simulink model "ball_impact"  (Simulink 8.1)
settings: Solver=ode4  SolverMode=SingleTasking  StartTime=0.0  StopTime=inf  FixedStep=0.0005  RelTol=1e-3
StartFcn:
  |  warndlg('Dexterit-E models cannot run under simulation. Please compile your model and run it from within Dexterit-E.');set_param(bdroot,'SimulationCommand','stop')
undefined symbols (not defined in the file or in its folder): CreateParameterTableGUI, slselsubs
libraries: xpclib x30, simulink x8, KINARM_general x3, KINARM_loads x2, Video x2, KINARM_EP_loads x1
(part 3 of 5)

== system ball_impact/Parameter Table Defn/events ==
  E_BALL_RELEASE;BALL_RELEASE;;Ball released at the slope top;;;none;; : Constant
  E_CONTACT_END;CONTACT_END;;Ball-hand contact ended;;;none;; : Constant  Value=3
  E_CONTACT_START;CONTACT_START;;Ball-hand contact started (pen greater than 0);;;none;; : Constant  Value=2
  E_HAND_LEFT_HOME;HAND_LEFT_HOME;;Hand left home before impact - trial aborted;;;error;; : Constant  Value=4
  Terminator{1..4} (4 alike) : Terminator
  wires:
  E_BALL_RELEASE;BALL_RELEASE;;Ball released at the slope top;;;none;;/1 -> Terminator1/1
  E_CONTACT_START;CONTACT_START;;Ball-hand contact started (pen greater than 0);;;none;;/1 -> Terminator2/1
  E_CONTACT_END;CONTACT_END;;Ball-hand contact ended;;;none;;/1 -> Terminator3/1
  E_HAND_LEFT_HOME;HAND_LEFT_HOME;;Hand left home before impact - trial aborted;;;error;;/1 -> Terminator4/1

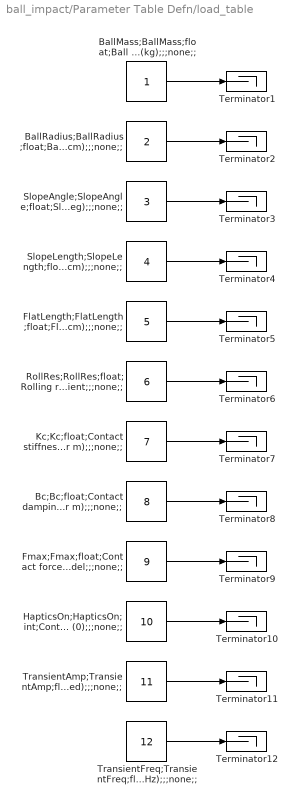
== system ball_impact/Parameter Table Defn/load_table ==
  BallMass;BallMass;float;Ball mass (kg);;;none;; : Constant
  BallRadius;BallRadius;float;Ball radius (cm);;;none;; : Constant  Value=2
  Bc;Bc;float;Contact damping (N s per m);;;none;; : Constant  Value=8
  FlatLength;FlatLength;float;Flat run-out length (cm);;;none;; : Constant  Value=5
  "Fmax;Fmax;float;Contact force clamp (N), also hard-clamped in the model;;;none;;" : Constant  Value=9
  HapticsOn;HapticsOn;int;Contact force on (1) or visual only (0);;;none;; : Constant  Value=10
  Kc;Kc;float;Contact stiffness (N per m);;;none;; : Constant  Value=7
  RollRes;RollRes;float;Rolling resistance coefficient;;;none;; : Constant  Value=6
  SlopeAngle;SlopeAngle;float;Slope angle (deg);;;none;; : Constant  Value=3
  SlopeLength;SlopeLength;float;Slope length (cm);;;none;; : Constant  Value=4
  Terminator{1..12} (12 alike) : Terminator
  TransientAmp;TransientAmp;float;Impact transient amplitude (N per unit impact speed);;;none;; : Constant  Value=11
  TransientFreq;TransientFreq;float;Impact transient frequency (Hz);;;none;; : Constant  Value=12
  wires:
  BallMass;BallMass;float;Ball mass (kg);;;none;;/1 -> Terminator1/1
  BallRadius;BallRadius;float;Ball radius (cm);;;none;;/1 -> Terminator2/1
  SlopeAngle;SlopeAngle;float;Slope angle (deg);;;none;;/1 -> Terminator3/1
  SlopeLength;SlopeLength;float;Slope length (cm);;;none;;/1 -> Terminator4/1
  FlatLength;FlatLength;float;Flat run-out length (cm);;;none;;/1 -> Terminator5/1
  RollRes;RollRes;float;Rolling resistance coefficient;;;none;;/1 -> Terminator6/1
  Kc;Kc;float;Contact stiffness (N per m);;;none;;/1 -> Terminator7/1
  Bc;Bc;float;Contact damping (N s per m);;;none;;/1 -> Terminator8/1
  "Fmax;Fmax;float;Contact force clamp (N), also hard-clamped in the model;;;none;;"/1 -> Terminator9/1
  HapticsOn;HapticsOn;int;Contact force on (1) or visual only (0);;;none;;/1 -> Terminator10/1
  TransientAmp;TransientAmp;float;Impact transient amplitude (N per unit impact speed);;;none;;/1 -> Terminator11/1
  TransientFreq;TransientFreq;float;Impact transient frequency (Hz);;;none;;/1 -> Terminator12/1

== system ball_impact/Parameter Table Defn/target_table ==
  Colour;Colour;colour;Target colour;;;none;; : Constant  Value=5
  LogRadius;LogRadius;float;Hand-in-target logical radius (cm);;;none;; : Constant  Value=4
  Terminator{1..5} (5 alike) : Terminator
  VisRadius;VisRadius;float;Drawn radius of the target circle (cm);;;none;; : Constant  Value=3
  col_x;X;float;X Position (cm) of the target relative to  local (0,0);;;none;; : Constant
  col_y;Y;float;Y Position (cm) of the target relative to  local (0,0);;;none;; : Constant  Value=2
  wires:
  col_x;X;float;X Position (cm) of the target relative to  local (0,0);;;none;;/1 -> Terminator1/1
  col_y;Y;float;Y Position (cm) of the target relative to  local (0,0);;;none;;/1 -> Terminator2/1
  VisRadius;VisRadius;float;Drawn radius of the target circle (cm);;;none;;/1 -> Terminator3/1
  LogRadius;LogRadius;float;Hand-in-target logical radius (cm);;;none;;/1 -> Terminator4/1
  Colour;Colour;colour;Target colour;;;none;;/1 -> Terminator5/1

== system ball_impact/Parameter Table Defn/task_definition ==
  INSTRUCTIONS= : Constant
  LOAD_FOR=EITHER : Constant  Value=2
  Terminator1 : Terminator
  Terminator2 : Terminator
  wires:
  INSTRUCTIONS=/1 -> Terminator1/1
  LOAD_FOR=EITHER/1 -> Terminator2/1

== system ball_impact/Parameter Table Defn/task_wide ==
  ApproachDir;ApproachDir;float;Ball approach direction (deg) with 90 = lateral from +X and 0 = toward body;;;none;; : Constant  Value=2
  HandRadius;HandRadius;float;Hand contact (paddle) radius (cm);;;none;; : Constant
  Terminator1 : Terminator
  Terminator2 : Terminator
  wires:
  HandRadius;HandRadius;float;Hand contact (paddle) radius (cm);;;none;;/1 -> Terminator1/1
  ApproachDir;ApproachDir;float;Ball approach direction (deg) with 90 = lateral from +X and 0 = toward body;;;none;;/1 -> Terminator2/1

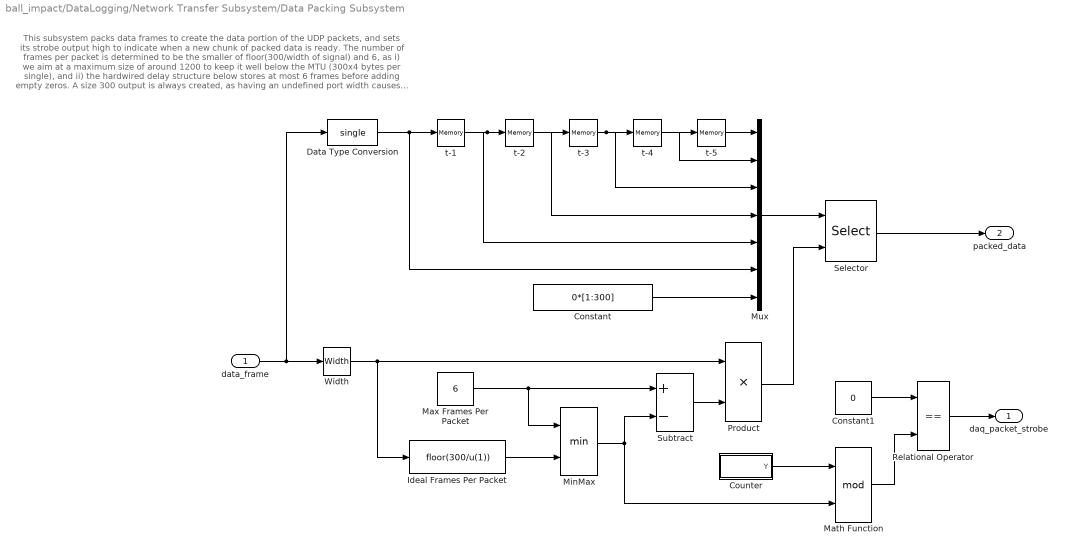
== system ball_impact/DataLogging/Network Transfer Subsystem/Data Packing Subsystem ==
  note: This subsystem packs data frames to create the data portion of the UDP packets, and sets its strobe output high to indicate when a
      | new chunk of packed data is ready. The number of frames per packet is determined to be the smaller of floor(300/width of signal)
      | and 6, as i) we aim at a maximum size of around 1200 to keep it well below the MTU (300x4 bytes per single), and ii) the hardwired
      | delay structure below stores at most 6 frames before adding empty zeros. A size 300 output is always created, as having an undefined
      | port width causes Simulink problems.
  data_frame : Inport
  Constant : Constant  Value=0*[1:300]  OutDataTypeStr=single
  Constant1 : Constant  Value=0
  Counter : Subsystem
  Data Type Conversion : DataTypeConversion  OutDataTypeStr=single  SaturateOnIntegerOverflow=on  RndMeth=Zero
  Ideal Frames Per Packet : Fcn  Expr=floor(300/u(1))
  Math Function : Math  Operator=mod  SaturateOnIntegerOverflow=on
  Max Frames Per Packet : Constant  Value=6
  MinMax : MinMax  Inputs=2
  Mux : Mux  Inputs=7
  Product : Product  RndMeth=Zero
  Relational Operator : RelationalOperator  Operator===  OutDataTypeStr=boolean
  Selector : Selector  IndexMode=Zero-based  IndexOptions=Starting index (port)  Indices=[1:300]  OutputSizes=[([([([([(300)])])])])]
  Subtract : Sum  Inputs=+-
  Width : Width
  t-{1..5} (5 alike) : Memory  InheritSampleTime=on
  daq_packet_strobe : Outport
  packed_data : Outport  Port=2
  wires:
  Ideal Frames Per Packet/1 -> MinMax/2
  Width/1 -> Ideal Frames Per Packet/1, Product/1
  Product/1 -> Selector/2
  Subtract/1 -> Product/2
  Max Frames Per Packet/1 -> MinMax/1, Subtract/1
  MinMax/1 -> Subtract/2, Math Function/2
  Constant/1 -> Mux/7
  Selector/1 -> packed_data/1
  Mux/1 -> Selector/1
  t-5/1 -> Mux/1
  Data Type Conversion/1 -> Mux/6, t-1/1
  t-3/1 -> Mux/3, t-4/1
  t-4/1 -> Mux/2, t-5/1
  t-2/1 -> Mux/4, t-3/1
  t-1/1 -> Mux/5, t-2/1
  Math Function/1 -> Relational Operator/2
  Constant1/1 -> Relational Operator/1
  Relational Operator/1 -> daq_packet_strobe/1
  Counter/1(Y) -> Math Function/1
  data_frame/1 -> Data Type Conversion/1, Width/1

== system ball_impact/DataLogging/Network Transfer Subsystem/UDP Send Subsystem ==
  packet_data : Inport
  Trigger : TriggerPort  TriggerType=function-call
  Counter Free-Running : simulink/Sources/Counter Free-Running  NumBits=32  tsamp=-1
  Pack : xpclib/UDP/Pack  datatypes={'single'}  byteAlign=1
  Send : xpclib/UDP/Send  ipAddress=192.168.0.1  ipPort=50000  localPort=50000  vblLen=off  sampletime=-1
  total_packets_sent : Outport  InitialOutput=0
  wires:
  packet_data/1 -> Pack/1
  Pack/1 -> Send/1
  Counter Free-Running/1 -> total_packets_sent/1

== system ball_impact/DataLogging/Poll Force Plates/plate1 ==
  send_packet : Inport
  gain : Inport  Port=2
  calib_matrix : Inport  Port=3
  ain_slope : Inport  Port=4
  ain_offset : Inport  Port=5
  orientation : Inport  Port=6
  zero_voltage : Inport  Port=7
  Enable : EnablePort
  Receive : xpclib/UDP/Receive  ipAddress=192.168.0.101  ipPort=53795  width=64  vblLen=off  sampletime=BKIN_STEP_TIME
  Send : xpclib/UDP/Send  ipAddress=192.168.0.101  ipPort=52360  localPort=53795  vblLen=off  sampletime=0.0005
  Terminator : Terminator
  parse packet 1 : MATLAB Function  TreatAsAtomicUnit=on
  Forces P1 : Outport
  Moments P1 : Outport  Port=2
  Timer P1 : Outport  Port=3
  wires:
  send_packet/1 -> Send/1
  parse packet 1/3(timer) -> Timer P1/1
  Receive/2 -> Terminator/1
  gain/1 -> parse packet 1/3(gain)
  Receive/1 -> parse packet 1/1(packet)
  calib_matrix/1 -> parse packet 1/2(calibration)
  parse packet 1/1(forces) -> Forces P1/1
  parse packet 1/2(moments) -> Moments P1/1
  ain_offset/1 -> parse packet 1/5(ain_offset)
  ain_slope/1 -> parse packet 1/4(ain_slope)
  orientation/1 -> parse packet 1/6(orientation)
  zero_voltage/1 -> parse packet 1/7(zero_voltage)

== system ball_impact/DataLogging/Poll Force Plates/plate2 ==
  send_packet : Inport
  gain : Inport  Port=2
  calib_matrix : Inport  Port=3
  ain_slope : Inport  Port=4
  ain_offset : Inport  Port=5
  orientation : Inport  Port=6
  zero_voltage : Inport  Port=7
  Enable : EnablePort
  Receive1 : xpclib/UDP/Receive  ipAddress=192.168.0.102  ipPort=53796  width=64  vblLen=off  sampletime=BKIN_STEP_TIME
  Send1 : xpclib/UDP/Send  ipAddress=192.168.0.102  ipPort=52360  localPort=53796  vblLen=off  sampletime=0.0005
  Terminator : Terminator
  parse packet 1 : MATLAB Function  TreatAsAtomicUnit=on
  Forces P1 : Outport
  Moments P1 : Outport  Port=2
  Timer P1 : Outport  Port=3
  wires:
  send_packet/1 -> Send1/1
  parse packet 1/3(timer) -> Timer P1/1
  Receive1/2 -> Terminator/1
  gain/1 -> parse packet 1/3(gain)
  Receive1/1 -> parse packet 1/1(packet)
  calib_matrix/1 -> parse packet 1/2(calibration)
  parse packet 1/1(forces) -> Forces P1/1
  parse packet 1/2(moments) -> Moments P1/1
  ain_offset/1 -> parse packet 1/5(ain_offset)
  ain_slope/1 -> parse packet 1/4(ain_slope)
  orientation/1 -> parse packet 1/6(orientation)
  zero_voltage/1 -> parse packet 1/7(zero_voltage)

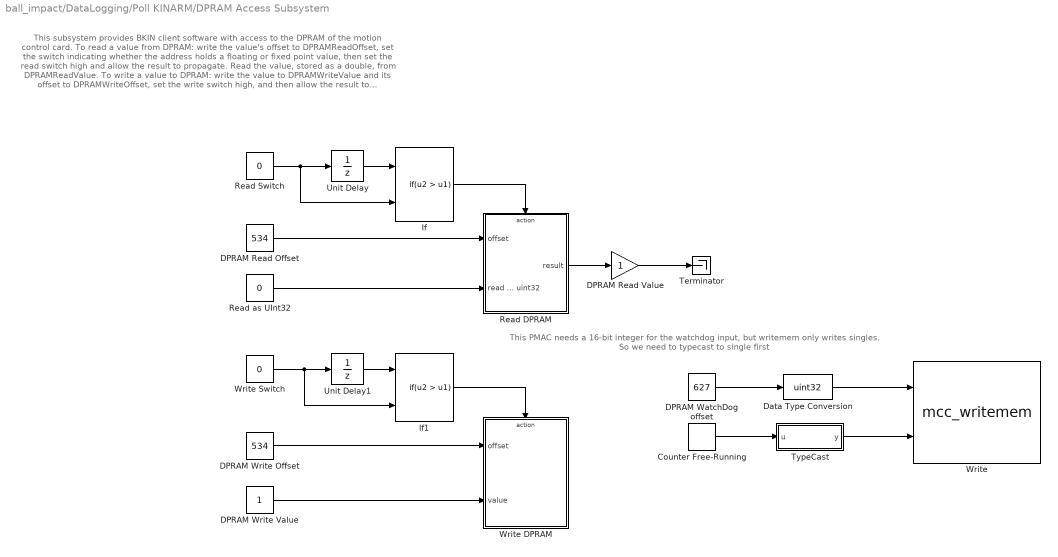
== system ball_impact/DataLogging/Poll KINARM/DPRAM Access Subsystem ==
  note: This PMAC needs a 16-bit integer for the watchdog input, but writemem
      | only writes singles.  So we need to typecast to single first
  note: This subsystem provides BKIN client software with access to the DPRAM of the motion control card.
      |
      | To read a value from DPRAM: write the value's offset to DPRAMReadOffset, set the switch indicating
      | whether the address holds a floating or fixed point value, then set the read switch high and allow the
      | result to propagate. Read the value, stored as a double, from DPRAMReadValue.
      |
      | To write a value to DPRAM: write the value to DPRAMWriteValue and its offset to DPRAMWriteOffset,
      | set the write switch high, and then allow the result to propagate. There is currently no option to write
      | values as UInt32s, akin to that for reading values.
      |
      | The default value for the offsets (0x216) is the lowest meaningful offset, the PLC switch variable.
  Counter Free-Running : simulink/Sources/Counter Free-Running  NumBits=16  tsamp=-1
  DPRAM Read Offset : Constant  Value=534  OutDataTypeStr=double
  DPRAM Read Value : Gain  SaturateOnIntegerOverflow=on  OutDataTypeStr=Inherit: Same as input  ParamDataTypeStr=Inherit: Same as input
  DPRAM WatchDog offset : Constant  Value=627  OutDataTypeStr=double
  DPRAM Write Offset : Constant  Value=534  OutDataTypeStr=double
  DPRAM Write Value : Constant
  Data Type Conversion : DataTypeConversion  OutDataTypeStr=uint32  SaturateOnIntegerOverflow=on  RndMeth=Zero
  If : If  NumInputs=2  IfExpression=u2 > u1  ShowElse=off
  If1 : If  NumInputs=2  IfExpression=u2 > u1  ShowElse=off
  Read DPRAM : Subsystem  TreatAsAtomicUnit=on
  Read Switch : Constant  Value=0
  Read as UInt32 : Constant  Value=0  OutDataTypeStr=double
  Terminator : Terminator
  TypeCast : MATLAB Function  TreatAsAtomicUnit=on
  Unit Delay : UnitDelay  SampleTime=-1
  Unit Delay1 : UnitDelay  SampleTime=-1
  Write : S-Function  Priority=6  FunctionName=mcc_writemem  EnableBusSupport=off
  Write DPRAM : Subsystem  TreatAsAtomicUnit=on
  Write Switch : Constant  Value=0
  wires:
  TypeCast/1(y) -> Write/2
  DPRAM Write Offset/1 -> Write DPRAM/1(offset)
  DPRAM Write Value/1 -> Write DPRAM/2(value)
  If1/1 -> Write DPRAM/Action
  Write Switch/1 -> Unit Delay1/1, If1/2
  DPRAM Read Value/1 -> Terminator/1
  Read DPRAM/1(result) -> DPRAM Read Value/1
  If/1 -> Read DPRAM/Action
  DPRAM Read Offset/1 -> Read DPRAM/1(offset)
  Read Switch/1 -> Unit Delay/1, If/2
  Unit Delay/1 -> If/1
  Unit Delay1/1 -> If1/1
  Read as UInt32/1 -> Read DPRAM/2(read as uint32)
  Data Type Conversion/1 -> Write/1
  DPRAM WatchDog offset/1 -> Data Type Conversion/1
  Counter Free-Running/1 -> TypeCast/1(u)

== system ball_impact/DataLogging/Poll KINARM/Force Sensor Control Subsystem ==
  note: This subsystem receives data from force sensors in the KINARM setup, and starts and stops the data transfer in response to changes in
      | the force sensor parameters in the system above. Each KINARM EP can have a force sensor, so there can currently be up to two in a
      | given setup. The force sensors transmit data over UDP, and parameters of the data transfer (such as the data rate and IP address) are
      | configured for each force sensor individually via a web interface they provide. BKIN preconfigures force sensors with IP addresses
      | 192.168.0.10-11, where the first address is given to the sensor for robot 1 and the second to that for robot 2.
  note: Each subsystem also handles the receiving of data from its particular sensor. When a sensor is indicated as present, the latest data from
      | its IP is unpacked and placed into a 1x6 array (zeros are explicitly specified when a sensor is indicated as not present). The arrays for
      | the individual sensors are combined into a 2x6 matrix, similar to how robot data is handled in the system above.
      |
      | Each packet received from a force sensor contains the following:
      |      sequence number [uint32]
      |      internal sequence number [uint32]
      |      system status code [uint32]
      |      x-axis force [int32]
      |      y-axis force [int32]
      |      z-axis force [int32]
      |      x-axis torque [int32]
      |      y-axis torque [int32]
      |      z-axis torque [int32]
      |
      | For more information, again see the ATI Net Interface guide.
  note: Each "force sensor x" subsystem here starts and stops the data transfer from its respective force sensor. When the input flag indicating
      | the presence (1: yes, 0: no) of a force sensor changes, the respective subsystem sends a command message via UDP to that force
      | sensor's IP address that starts or stops the data transfer accordingly. For details about the structure of the command message, see the
      | ATI Net Interface guide.
      |
      | Note that the default setting for all force sensors is 1, for "present", in the system above. This is done so that whenever BKIN's client
      | software applies hardware settings to a task program, it must first lower all force sensor flags and then raise those for whichever sensors
      | are present again. This forces all sensors off in case they were not stopped properly by a previous task. This would not stop data that
      | had been transmitted from being received, so when a force sensor is marked as not present the data is zeroed explicitly.
  Robot 1 Force Sensor : Inport
  Robot 2 Force Sensor : Inport  Port=2
  Force Sensor 1 Subsystem : Subsystem
  Force Sensor 2 Subsystem : Subsystem
  Mux8 : Mux  Inputs=2
  Force Sensor Data : Outport
  wires:
  Robot 1 Force Sensor/1 -> Force Sensor 1 Subsystem/1(Force Sensor 1 Present)
  Robot 2 Force Sensor/1 -> Force Sensor 2 Subsystem/1(Force Sensor 2 Present)
  Force Sensor 1 Subsystem/1(Out1) -> Mux8/1
  Force Sensor 2 Subsystem/1(Out1) -> Mux8/2
  Mux8/1 -> Force Sensor Data/1

== system ball_impact/DataLogging/Poll KINARM/Terminators for Gotos ==
  Terminator{,1..4} (5 alike) : Terminator
  wires:
  [primary_encoder_data] -> Terminator/1
  [robot1_motor_parameters] -> Terminator1/1
  [robot2_motor_parameters] -> Terminator2/1
  [robot1_calibration_parameters] -> Terminator3/1
  [robot2_calibration_parameters] -> Terminator4/1

== system ball_impact/DataLogging/Network Transfer Subsystem/Data Packing Subsystem/Counter ==
  Constant : Constant
  Sum : Sum  Inputs=|++  SaturateOnIntegerOverflow=on
  Unit Delay : UnitDelay  SampleTime=-1
  Y : Outport
  wires:
  Constant/1 -> Sum/2
  Sum/1 -> Unit Delay/1, Y/1
  Unit Delay/1 -> Sum/1

== system ball_impact/DataLogging/Poll KINARM/DPRAM Access Subsystem/Read DPRAM ==
  offset : Inport
  read as uint32 : Inport  Port=2
  Action Port : ActionPort
  Data Type Conversion : DataTypeConversion  OutDataTypeStr=uint32  SaturateOnIntegerOverflow=on  RndMeth=Zero
  Data Type Conversion1 : DataTypeConversion  OutDataTypeStr=double  SaturateOnIntegerOverflow=on  RndMeth=Zero
  Data Type Conversion2 : DataTypeConversion  OutDataTypeStr=uint32  SaturateOnIntegerOverflow=on  RndMeth=Zero
  Mux : Mux  Inputs=2
  Read : S-Function  Priority=6  FunctionName=mcc_readmem  EnableBusSupport=off
  result : Outport
  wires:
  Data Type Conversion/1 -> Mux/1
  Data Type Conversion1/1 -> result/1
  Read/1 -> Data Type Conversion1/1
  offset/1 -> Data Type Conversion/1
  read as uint32/1 -> Data Type Conversion2/1
  Data Type Conversion2/1 -> Mux/2
  Mux/1 -> Read/1

== system ball_impact/DataLogging/Poll KINARM/DPRAM Access Subsystem/Write DPRAM ==
  offset : Inport
  value : Inport  Port=2
  Action Port : ActionPort
  Data Type Conversion : DataTypeConversion  OutDataTypeStr=uint32  SaturateOnIntegerOverflow=on  RndMeth=Zero
  Data Type Conversion1 : DataTypeConversion  OutDataTypeStr=single  SaturateOnIntegerOverflow=on  RndMeth=Zero
  Write : S-Function  Priority=6  FunctionName=mcc_writemem  EnableBusSupport=off
  wires:
  Data Type Conversion1/1 -> Write/2
  Data Type Conversion/1 -> Write/1
  offset/1 -> Data Type Conversion/1
  value/1 -> Data Type Conversion1/1

== system ball_impact/DataLogging/Poll KINARM/Force Sensor Control Subsystem/Force Sensor 1 Subsystem ==
  Force Sensor 1 Present : Inport
  Byte Reversal : xpclib/UDP/Byte Reversal  numInp=1
  Byte Reversal1 : xpclib/UDP/Byte Reversal  numInp=1
  Constant : Constant  Value=zeros(1, 7);  OutDataTypeStr=double
  Create timestamp : MATLAB Function  TreatAsAtomicUnit=on
  Data Type Conversion : DataTypeConversion
  Detect Change : simulink/Logic and Bit Operations/Detect Change  vinit=1  InputProcessing=Inherited  OutDataTypeStr=uint8
  If Action Subsystem : Subsystem  TreatAsAtomicUnit=on
  Mux : Mux  Inputs=2
  Receive from Robot 1 Force Sensor : xpclib/UDP/Receive  ipAddress=192.168.0.10  ipPort=51000  width=36  vblLen=off  sampletime=BKIN_STEP_TIME
  Switch : Switch  Criteria=u2 > Threshold
  Terminator : Terminator
  Unpack : xpclib/UDP/Unpack  dimensions={3, 6}  datatypes={'uint32', 'int32'}  byteAlign=1
  Out1 : Outport
  wires:
  Receive from Robot 1 Force Sensor/1 -> Unpack/1
  Receive from Robot 1 Force Sensor/2 -> Terminator/1
  Force Sensor 1 Present/1 -> Switch/2, If Action Subsystem/1(In1), Detect Change/1
  Constant/1 -> Switch/3
  Switch/1 -> Out1/1
  Unpack/2 -> Byte Reversal/1
  Unpack/1 -> Byte Reversal1/1
  Byte Reversal/1 -> Data Type Conversion/1
  Detect Change/1 -> If Action Subsystem/Enable
  Create timestamp/1(timestamp_out) -> Mux/2
  Data Type Conversion/1 -> Mux/1
  Mux/1 -> Switch/1
  Byte Reversal1/1 -> Create timestamp/1(times_in)

== system ball_impact/DataLogging/Poll KINARM/Force Sensor Control Subsystem/Force Sensor 2 Subsystem ==
  Force Sensor 2 Present : Inport
  Byte Reversal : xpclib/UDP/Byte Reversal  numInp=1
  Byte Reversal1 : xpclib/UDP/Byte Reversal  numInp=1
  Constant1 : Constant  Value=zeros(1, 7);  OutDataTypeStr=double
  Create timestamp : MATLAB Function  TreatAsAtomicUnit=on
  Data Transfer Start Subsystem : Subsystem  TreatAsAtomicUnit=on
  Data Type Conversion1 : DataTypeConversion
  Detect Change : simulink/Logic and Bit Operations/Detect Change  vinit=1  InputProcessing=Inherited  OutDataTypeStr=uint8
  Mux : Mux  Inputs=2
  Receive from Robot 2 Force Sensor : xpclib/UDP/Receive  ipAddress=192.168.0.11  ipPort=51001  width=36  vblLen=off  sampletime=BKIN_STEP_TIME
  Switch1 : Switch  Criteria=u2 > Threshold
  Terminator1 : Terminator
  Unpack1 : xpclib/UDP/Unpack  dimensions={3, 6}  datatypes={'uint32', 'int32'}  byteAlign=1
  Out1 : Outport
  wires:
  Receive from Robot 2 Force Sensor/1 -> Unpack1/1
  Receive from Robot 2 Force Sensor/2 -> Terminator1/1
  Force Sensor 2 Present/1 -> Switch1/2, Data Transfer Start Subsystem/1(In2), Detect Change/1
  Constant1/1 -> Switch1/3
  Switch1/1 -> Out1/1
  Unpack1/2 -> Byte Reversal/1
  Byte Reversal/1 -> Data Type Conversion1/1
  Detect Change/1 -> Data Transfer Start Subsystem/Enable
  Unpack1/1 -> Byte Reversal1/1
  Data Type Conversion1/1 -> Mux/1
  Create timestamp/1(timestamp_out) -> Mux/2
  Mux/1 -> Switch1/1
  Byte Reversal1/1 -> Create timestamp/1(times_in)

== system ball_impact/DataLogging/Poll KINARM/Force Sensor Control Subsystem/Force Sensor 1 Subsystem/If Action Subsystem ==
  In1 : Inport
  Enable : EnablePort
  Byte Reversal : xpclib/UDP/Byte Reversal  numInp=1
  Byte Reversal1 : xpclib/UDP/Byte Reversal  numInp=1
  Byte Reversal2 : xpclib/UDP/Byte Reversal  numInp=1
  Constant : Constant  Value=4660  OutDataTypeStr=uint16
  Constant1 : Constant  Value=0  OutDataTypeStr=uint32
  Constant2 : Constant  Value=0  OutDataTypeStr=uint16
  Constant3 : Constant  Value=2  OutDataTypeStr=uint16
  Pack : xpclib/UDP/Pack  datatypes={'uint16', 'uint16', 'uint32'}  byteAlign=1
  Send : xpclib/UDP/Send  ipAddress=192.168.0.10  ipPort=49152  localPort=51000  vblLen=off  sampletime=-1
  Switch : Switch  Criteria=u2 > Threshold
  wires:
  In1/1 -> Switch/2
  Constant/1 -> Byte Reversal1/1
  Constant1/1 -> Byte Reversal2/1
  Constant3/1 -> Switch/1
  Constant2/1 -> Switch/3
  Switch/1 -> Byte Reversal/1
  Pack/1 -> Send/1
  Byte Reversal1/1 -> Pack/1
  Byte Reversal/1 -> Pack/2
  Byte Reversal2/1 -> Pack/3

== system ball_impact/DataLogging/Poll KINARM/Force Sensor Control Subsystem/Force Sensor 2 Subsystem/Data Transfer Start Subsystem ==
  In2 : Inport
  Enable : EnablePort
  Byte Reversal : xpclib/UDP/Byte Reversal  numInp=1
  Byte Reversal1 : xpclib/UDP/Byte Reversal  numInp=1
  Byte Reversal2 : xpclib/UDP/Byte Reversal  numInp=1
  Constant : Constant  Value=4660  OutDataTypeStr=uint16
  Constant1 : Constant  Value=0  OutDataTypeStr=uint32
  Constant2 : Constant  Value=0  OutDataTypeStr=uint16
  Constant3 : Constant  Value=2  OutDataTypeStr=uint16
  Pack : xpclib/UDP/Pack  datatypes={'uint16', 'uint16', 'uint32'}  byteAlign=1
  Send : xpclib/UDP/Send  ipAddress=192.168.0.11  ipPort=49152  localPort=51001  vblLen=off  sampletime=-1
  Switch : Switch  Criteria=u2 > Threshold
  wires:
  In2/1 -> Switch/2
  Constant/1 -> Byte Reversal1/1
  Constant1/1 -> Byte Reversal/1
  Constant3/1 -> Switch/1
  Constant2/1 -> Switch/3
  Switch/1 -> Byte Reversal2/1
  Pack/1 -> Send/1
  Byte Reversal/1 -> Pack/3
  Byte Reversal1/1 -> Pack/1
  Byte Reversal2/1 -> Pack/2

== stateflow chart Trial_Control ==
  state WAIT_HOME
    entry:
    logging_enable = 1;
    target_row = Trial_Protocol[HomeTarget];
    target_state = 1;
    load_row = Trial_Protocol[Load];
    ball_row = Trial_Protocol[BallTarget];
    phase = 0;
    event_code = 0;
  state HOLD
    entry:
    TimeInterval = Trial_Protocol[HoldTime];
  state RELEASE_WAIT
    entry:
    phase = 1;
    TimeInterval = delay_fb;
  state ROLLING
    entry:
    phase = 2;
    event_code = E_BALL_RELEASE;
    TimeInterval = timeout_fb;
  state CONTACT
    entry:
    event_code = E_CONTACT_START;
  state POST_IMPACT
    entry:
    event_code = E_CONTACT_END;
  state ABORT_LEAVE
    entry:
    event_code = E_HAND_LEFT_HOME;
  state EndOfTrial
    entry:
    logging_enable = 0;
    target_state = 0;
    phase = 0;
    send(e_Trial_End);
  RELEASE_WAIT -> WAIT_HOME [order 2] : [HandInTarget[target_row] == 0]
  HOLD -> WAIT_HOME [order 2] : [HandInTarget[target_row] == 0]
  WAIT_HOME -> HOLD : [HandInTarget[target_row] == 1]
  (default) -> WAIT_HOME
  EndOfTrial -> WAIT_HOME : after(1000, e_clk)
  HOLD -> RELEASE_WAIT [order 1] : after(TimeInterval, e_clk)
  RELEASE_WAIT -> ROLLING [order 1] : after(TimeInterval, e_clk)
  ROLLING -> ABORT_LEAVE [order 2] : [HandInTarget[target_row] == 0]
  ABORT_LEAVE -> EndOfTrial : after(10, e_clk)
  ROLLING -> EndOfTrial [order 3] : after(TimeInterval, e_clk)
  ROLLING -> CONTACT [order 1] : [pen_fb > 0]
  CONTACT -> POST_IMPACT : after(5, e_clk)[pen_fb <= 0]
  POST_IMPACT -> CONTACT [order 1] : [pen_fb > 0]
  POST_IMPACT -> EndOfTrial [order 3] : after(2500, e_clk)
  POST_IMPACT -> EndOfTrial [order 2] : after(300, e_clk)[speed_fb < 0.02]
  data: Trial_Protocol input double; HandInTarget input double; logging_enable output double; target_row output double; target_state output double; TimeInterval local double; pen_fb input double; speed_fb input double; event_code output double; phase output double; load_row output double; ball_row output double; delay_fb input double; timeout_fb input double
  events: e_clk input RISING_EDGE_EVENT; e_ExitTrialNow input EITHER_EDGE_EVENT; e_Trial_End output EITHER_EDGE_EVENT

== matlab function Ball_Engine ==
  data: phase input double; vcodes output double; home_row input double; ball_row input double; load_row input double; KINdata input double; Load_Table input double; Target_Table input double; Task_Wide input double; TP_Table input double; tp_row input double; seed input double; hand_in input double; hand_forces output double; ball_log output double; pen_out output double; speed_out output double; delay_ms output double; timeout_ms output double
function [vcodes, hand_forces, ball_log, pen_out, speed_out, delay_ms, timeout_ms] = ball_engine(phase, home_row, ball_row, load_row, KINdata, Load_Table, Target_Table, Task_Wide, TP_Table, tp_row, seed, hand_in) %#codegen
%BALL_ENGINE Ball physics, penalty contact force, and ball/slope VCODEs.
%
% Runs every 1 ms. The Trial_Control chart sequences the trial and sets:
%   phase 0 = no ball (reset), 1 = ball parked at slope top, 2 = physics live.
% The ball is constrained to the line from the slope top (Target Table row
% ball_row) toward the home target (row home_row): gravity component
% (5/7)*g*sin(theta) acts along it while the path distance s < SlopeLength,
% rolling resistance -RollRes*g*sign(v) always. Contact with the hand disk is
% penalty-based: pen = BallRadius + HandRadius - |p_hand - p_ball|, force
% clamp(Kc*pen + Bc*dpen/dt, 0, Fmax) along the ball-to-hand normal, plus a
% decaying TransientFreq sinusoid for the first 30 ms of each new contact.
% The reaction decelerates the ball (bounce); HapticsOn=0 zeroes the commanded
% force but keeps the visual bounce. Fmax is hard-clamped at 45 N.
%
% Units: Target Table and lengths in the Load Table are cm (converted to m
% here); KINdata hand position/velocity are m, m/s, global frame; forces N.

persistent s v prev_pen t_contact have_contact initd rngstate
if isempty(initd)
    s = 0; v = 0; initd = 1;
    prev_pen = [0 0]; t_contact = [1e9 1e9]; have_contact = [0 0];
    rngstate = mod(abs(seed), 4294967296);
    if rngstate <= 0; rngstate = 12345; end
end

dt = 0.001;
g  = 9.81;

% ---- per-trial timing for the chart (sampled by Stateflow at state entry).
% R2013a chart codegen cannot lower rand()/boolean arithmetic, so the random
% release delay and the zero-timeout guard are computed here instead. LCG
% seeded from Dexterit-E's 'seed' tag, so the protocol seed option holds.
rngstate = mod(1664525 * rngstate + 1013904223, 4294967296);
u = rngstate / 4294967296;
tr = max(1, min(100, round(tp_row)));
dmin = TP_Table(tr, 5);
dmax = TP_Table(tr, 6);
if dmax > dmin
    delay_ms = dmin + (dmax - dmin) * u;
else
    delay_ms = dmin;
end
if delay_ms < 0; delay_ms = 0; end
timeout_ms = TP_Table(tr, 7);
if timeout_ms <= 0; timeout_ms = 10000; end

vcodes      = zeros(9, 70);
hand_forces = zeros(4, 1);

% ---- parameters ------------------------------------------------------------
hr = max(1, min(32, round(home_row)));
br = max(1, min(32, round(ball_row)));
lr = max(1, min(20, round(load_row)));

m_b    = Load_Table(lr, 1);
r_b    = Load_Table(lr, 2) * 0.01;
theta  = Load_Table(lr, 3) * pi / 180;
Lslope = Load_Table(lr, 4) * 0.01;
crr    = Load_Table(lr, 6);
kc     = Load_Table(lr, 7);
bc     = Load_Table(lr, 8);
Fmax   = Load_Table(lr, 9);
hapt   = Load_Table(lr, 10);
tamp   = Load_Table(lr, 11);
tfreq  = Load_Table(lr, 12);

% Defaults so an all-zero Load row stays safe and visible
if m_b <= 0;    m_b = 0.2;     end
if r_b <= 0;    r_b = 0.03;    end
if Lslope <= 0; Lslope = 0.20; end
if kc <= 0;     kc = 2000;     end
if Fmax <= 0;   Fmax = 20;     end
if Fmax > 45;   Fmax = 45;     end   % hardware envelope hard clamp
if tfreq < 50;  tfreq = 150;   end

r_h = Task_Wide(1) * 0.01;
if r_h <= 0; r_h = 0.02; end

% ---- geometry (global metres; Target_Table is global cm on the target) -----
tx  = Target_Table(br, 1) * 0.01;
ty  = Target_Table(br, 2) * 0.01;
hx0 = Target_Table(hr, 1) * 0.01;
hy0 = Target_Table(hr, 2) * 0.01;
dx = hx0 - tx; dy = hy0 - ty;
dd = sqrt(dx*dx + dy*dy);
if dd < 1e-6; dd = 1; end
ux = dx / dd; uy = dy / dd;

% ---- hand state: BOTH hands can strike the ball (row 1 = robot 1, row 2 =
% robot 2; an absent robot reads position (0,0), far from the track, so its
% penetration never goes positive) ---------------------------------------
hpx = [KINdata(1, 23) KINdata(2, 23)];
hpy = [KINdata(1, 24) KINdata(2, 24)];

% ---- physics ----------------------------------------------------------------
Fxh = [0 0]; Fyh = [0 0]; pen = 0;
if phase < 1.5
    % phase 0: hidden/reset. phase 1: parked at slope top.
    s = 0; v = 0;
    prev_pen = [0 0]; have_contact = [0 0]; t_contact = [1e9 1e9];
else
    a = 0;
    if s < Lslope
        a = a + (5/7) * g * sin(theta);   % downhill along +u while on the slope
    end
    if v > 1e-4
        a = a - crr * g;
    elseif v < -1e-4
        a = a + crr * g;
    end

    bxp = tx + ux * s; byp = ty + uy * s;
    for h = 1:2
        rx = hpx(h) - bxp; ry = hpy(h) - byp;
        dist = sqrt(rx*rx + ry*ry);
        if dist < 1e-6; dist = 1e-6; end
        penh = (r_b + r_h) - dist;

        if penh > 0
            dpen = (penh - prev_pen(h)) / dt;
            fmag = kc * penh + bc * dpen;
            if fmag < 0; fmag = 0; end
            if have_contact(h) == 0
                have_contact(h) = 1;
                t_contact(h) = 0;    % new contact: restart transient
            end
            if t_contact(h) < 0.03 && tamp > 0
                fmag = fmag + tamp * exp(-t_contact(h) / 0.01) * sin(2 * pi * tfreq * t_contact(h));
                if fmag < 0; fmag = 0; end
            end
            if fmag > Fmax; fmag = Fmax; end
            nx = rx / dist; ny = ry / dist;
            Fxh(h) = fmag * nx; Fyh(h) = fmag * ny;
            % equal and opposite on the ball, projected on the rail
            a = a - (Fxh(h) * ux + Fyh(h) * uy) / m_b;
        else
            have_contact(h) = 0;
        end
        t_contact(h) = t_contact(h) + dt;
        prev_pen(h) = penh;
        if penh > pen; pen = penh; end
    end

    v = v + a * dt;
    s = s + v * dt;
    if s < 0
        s = 0; v = -0.2 * v;   % cannot leave the top of the slope
    end
end

% ---- haptics gate (visual bounce unaffected) --------------------------------
if hapt < 0.5
    Fxh = [0 0]; Fyh = [0 0];
end
hand_forces(1) = Fxh(1); hand_forces(2) = Fyh(1);
hand_forces(3) = Fxh(2); hand_forces(4) = Fyh(2);
Fx = Fxh(1) + Fxh(2);               % total contact force, for the log
Fy = Fyh(1) + Fyh(2);

% ---- VCODEs (subject display mock, lateral slope) ---------------------------
% Rows: 1 flat run-out (darkest), 2-5 slope bar (4 shaded segments, lightest
% at the top), 6 slope-foot tick, 7 home ring (hollow; green when the hand is
% inside the home target), 8 ball (yellow; flashes white during contact),
% 9 ball highlight. Track and ring are always visible; the ball exists only
% during RELEASE_WAIT/ROLLING (phase > 0). The home target's filled circle is
% suppressed in the protocol via VisRadius = 0 (LogRadius still defines the
% logical zone and this ring's radius).
show = 0;
if phase > 0.5; show = 1; end

ringr = Target_Table(hr, 4) * 0.01;
if ringr <= 0; ringr = 0.015; end

footx = tx + ux * Lslope;  footy = ty + uy * Lslope;
flat_len = (dd - ringr - 0.005) - Lslope;
if flat_len < 0; flat_len = 0; end

barw = 0.02;

vcodes(1, 1)  = 4;                 % flat run-out: foot -> ring edge
vcodes(1, 2)  = 1;
vcodes(1, 3)  = footx;
vcodes(1, 4)  = footy;
vcodes(1, 5)  = 3158064;           % 0x303030
vcodes(1, 6)  = 3158064;
vcodes(1, 7)  = barw;
vcodes(1, 9)  = 100;
vcodes(1, 10) = ux * flat_len;
vcodes(1, 11) = uy * flat_len;

segc = [5921370 5197647 4473924 3750201];   % 0x5A5A5A -> 0x393939
seg  = Lslope / 4;
for i = 1:4
    vcodes(1+i, 1)  = 4;
    vcodes(1+i, 2)  = 1;
    vcodes(1+i, 3)  = tx + ux * seg * (i - 1);
    vcodes(1+i, 4)  = ty + uy * seg * (i - 1);
    vcodes(1+i, 5)  = segc(i);
    vcodes(1+i, 6)  = segc(i);
    vcodes(1+i, 7)  = barw;
    vcodes(1+i, 9)  = 100;
    vcodes(1+i, 10) = ux * seg;
    vcodes(1+i, 11) = uy * seg;
end

px = -uy; py = ux;                 % slope-foot tick, perpendicular to rail
vcodes(6, 1)  = 4;
vcodes(6, 2)  = 1;
vcodes(6, 3)  = footx - px * 0.014;
vcodes(6, 4)  = footy - py * 0.014;
vcodes(6, 5)  = 13158600;          % 0xC8C8C8
vcodes(6, 6)  = 13158600;
vcodes(6, 7)  = 0.0025;
vcodes(6, 9)  = 100;
vcodes(6, 10) = px * 0.028;
vcodes(6, 11) = py * 0.028;

ringc = 16777215;                  % white; green while the hand is at home
if hand_in(hr) > 0.5
    ringc = 3066993;               % 0x2ECC71
end
vcodes(7, 1)  = 1;                 % home ring (hollow circle)
vcodes(7, 2)  = 1;
vcodes(7, 3)  = hx0;
vcodes(7, 4)  = hy0;
vcodes(7, 5)  = 16777216;          % no fill
vcodes(7, 6)  = ringc;
vcodes(7, 7)  = 0.003;
vcodes(7, 9)  = 100;
vcodes(7, 10) = ringr;

bx = tx + ux * s; by = ty + uy * s;
ballc = 16106818;                  % 0xF5C542 yellow
hilc  = 16774080;                  % 0xFFF3C0 warm white highlight
if pen > 0
    ballc = 16777215;              % contact flash: white ball,
    hilc  = 16113824;              % 0xF5E0A0 pale yellow highlight
end
vcodes(8, 1)  = 1;                 % ball
vcodes(8, 2)  = show;
vcodes(8, 3)  = bx;
vcodes(8, 4)  = by;
vcodes(8, 5)  = ballc;
vcodes(8, 6)  = -2147483648;       % no stroke colour
vcodes(8, 7)  = 0;
vcodes(8, 9)  = 100;
vcodes(8, 10) = r_b;

vcodes(9, 1)  = 1;                 % highlight, upper-left of the ball centre
vcodes(9, 2)  = show;
vcodes(9, 3)  = bx - 0.35 * r_b;
vcodes(9, 4)  = by + 0.35 * r_b;
vcodes(9, 5)  = hilc;
vcodes(9, 6)  = -2147483648;
vcodes(9, 7)  = 0;
vcodes(9, 9)  = 100;
vcodes(9, 10) = 0.3 * r_b;

if s > dd + 0.6
    vcodes(8, 2) = 0;              % rolled far out of the scene
    vcodes(9, 2) = 0;
end

ball_log  = [bx; by; v; pen; Fx; Fy; phase; s];
pen_out   = pen;
speed_out = v;
if speed_out < 0; speed_out = -speed_out; end

== matlab function GUI Control/Preview Targets Subsystem/Create Target Vector ==
  settings: fimath=|
      | fimath(...
      | 'RoundMode', 'floor',...
      | 'OverflowMode', 'wrap',...
      | 'ProductMode', 'KeepLSB', 'ProductWordLength', 32,...
      | 'SumMode', 'KeepLSB', 'SumWordLength', 32,...
      | 'CastBeforeSum', false)
  data: target_table input double; target_type input double; target_vector output double; xy_column_indices input double; attrib_column_indices input double; target_vector_length output double
function [target_vector, target_vector_length]= create_target_vector(target_table, target_type, xy_column_indices, attrib_column_indices)

% Assemble the target vector for reading by the GUI. The vector consists of n entries back-to-back,
% where n is the number of rows in the target table, and each entry consists of
%
%   target type, x position, y position, visual attribute values, logical attribute values
%
% for a target, where all values are taken out of the target table and processed so that they are ready
% to be used by the GUI. This is kind of a compressed version of the process of creating a target using
% Show_Target block -> VCODE -> Process_Video_CMD block.
%
% The visual and logical attributes are the target type-specific information corresponding to the visual
% and logical versions of that target. Distances and rotations are converted from cm and degrees, as they
% are specified in the GUI, to um and and urads. For more information on how these are defined for each 
% target type, refer to the mask help for this block or for the Show_Target block.

% Note the number of attribute columns based on the target type.
num_attributes = 1;

if target_type == 1
    num_attributes = 1;
elseif target_type == 2 || target_type == 3 || target_type == 4
    num_attributes = 3;
elseif target_type == 5
    num_attributes = 4;
end

target_entry_size = num_attributes * 2 + 3;  % size of type, x,y position, and all attributes
table_size = size(target_table);

% Set the vector length to the maximum that might be required, as it has to be constant at build time.
target_vector_length = table_size(1) * 11;
target_vector = zeros(1, target_vector_length);

indices = attrib_column_indices;

% For each target, set...
for i = 1:table_size(1)
    start_index = (i-1) * target_entry_size + 1;
    
    target_vector(start_index) = target_type;  % target type
    
    target_vector(start_index+1) = target_table(i, xy_column_indices(1)) * 0.01;  % x position (m)
    target_vector(start_index+2) = target_table(i, xy_column_indices(2)) * 0.01;  % y position (m)
    
    % For each vector of visual and logical column indices...
    for j = 1:2
        attrib_start = start_index + 3 + (j-1) * num_attributes;
        
        % Copy circle attributes: radius (m).
        if target_type == 1
            target_vector(attrib_start) = target_table(i, indices(j, 1)) * 0.01;
    
        % Copy ellipse attributes: major radius (m), minor radius (m), rotation (degrees).
        elseif target_type == 2
            if indices(j, 1) == 0 || indices(j, 2) == 0
                target_vector(attrib_start) = 0.0;
                target_vector(attrib_start+1) = 0.0;
            else
                target_vector(attrib_start) = target_table(i, indices(j, 1)) * 0.01;
                target_vector(attrib_start+1) = target_table(i, indices(j, 2)) * 0.01;
            end
    
            if indices(j, 3) == 0
                target_vector(attrib_start+2) = 0.0;
            else
                target_vector(attrib_start+2) = mod(target_table(i, indices(j, 3)), 360) * pi / 180.0;
            end
        
        % Copy rectangle attributes: length (m), height (m), rotation (degrees).
        % This amounts to the same procedure as for an ellipse.
        elseif target_type == 3
            if indices(j, 1) == 0 || indices(j, 2) == 0
                target_vector(attrib_start) = 0.0;
                target_vector(attrib_start+1) = 0.0;
            else
                target_vector(attrib_start) = target_table(i, indices(j, 1)) * 0.01;
                target_vector(attrib_start+1) = target_table(i, indices(j, 2)) * 0.01;
            end
            
            if indices(j, 3) == 0
                target_vector(attrib_start+2) = 0.0;
            else
                target_vector(attrib_start+2) = mod(target_table(i, indices(j, 3)), 360) * pi / 180.0;
            end
            
    	% Copy line attributes: relative endpoint x coordinate (m), relative endpoint y coordinate (m), width
        elseif target_type == 4
            if (indices(j, 1) == 0 && indices(j, 2) == 0) || indices(j, 3) == 0
                target_vector(attrib_start) = 0.0;
                target_vector(attrib_start+1) = 0.0;
                target_vector(attrib_start+2) = 0.0;
            else
                target_vector(attrib_start) = target_table(i, indices(j, 1)) * 0.01;
                target_vector(attrib_start+1) = target_table(i, indices(j, 2)) * 0.01;
                
                if indices(j, 3) < 0
                    target_vector(attrib_start+2) = 0.001;
                else
                    target_vector(attrib_start+2) = target_table(i, indices(j, 3)) * 0.01;
                end
            end
            
        % Copy triangle attributes: length (m), height (m), peak offset (m), rotation (degrees).
        elseif target_type == 5
            if indices(j, 1) == 0
                target_vector(attrib_start) = 0.0;
            else
                target_vector(attrib_start) = target_table(i, indices(j, 1)) * 0.01;
            end
    
            if indices(j, 2) == 0  % create an equilateral triangle if no height column is specified
                target_vector(attrib_start+1) = target_table(i, indices(j, 1)) * sin(pi/3.0) * 0.01;
                target_vector(attrib_start+2) = 0.0;
            else
                target_vector(attrib_start+1) = target_table(i, indices(j, 2)) * 0.01;
                target_vector(attrib_start+2) = target_table(i, indices(j, 3)) * 0.01;
            end
            
            if indices(j, 4) == 0
                target_vector(attrib_start+3) = 0.0;
            else
                target_vector(attrib_start+3) = mod(target_table(i, indices(j, 4)), 360) * pi / 180.0;
            end
        end
    end
end

== stateflow chart DataLogging/Network Transfer Subsystem/Send Control Machine ==
  state SendControlMachine [parallel]
    settings: executionOrder=2
    state Idle
      // Wait to acquire a new packet to send.
    state SendPacket/
      CopyOutput(queue_tail); // copy oldest packet in packet_queue to output
      data_out[2] = queue_size;
      data_out[3] = total_timeouts;
      outstanding_packet_index = data_out[0];
      e_send;
    state WaitForACK/
      // Wait for an acknowledgement of the sent packet.
    (default) -> Idle
    (junction 90) -> Idle [order 1] : [queue_head == queue_tail]
    (junction 91) -> (junction 90) : [ack_packet_index == outstanding_packet_index]
        | { queue_tail = fmod(queue_tail + 1, packet_queue_sz); }
    (junction 90) -> SendPacket [order 2] : [queue_head != queue_tail]
    Idle -> SendPacket : [queue_head != queue_tail]
    SendPacket -> (junction 91) [order 1] : [ack_received_flag == 1]
    WaitForACK -> (junction 91) [order 2] : [ack_received_flag == 1]
    SendPacket -> WaitForACK [order 2]
    (junction 92) -> SendPacket [order 2]
    (junction 92) -> SendPacket [order 1] : [is_task_running == 1]
        | {total_timeouts++;}
    WaitForACK -> (junction 92) [order 1] : after(10, e_clock)  // resend after 10ms
  note: A trailing zero is added for safety, as the end of a packet is denoted
      | by a zero in place of the timestamp for a data frame. If the frame size is
      | such that the packet is completely filled, this zero would not be present
      | without this explicit addition.
  state UpdatePacketQueue [parallel]
    settings: executionOrder=1
    state AddPacketToQueue
    (default) -> AddPacketToQueue
    AddPacketToQueue -> (junction 104) : e_data_ready_strobe
        | {
        | // Prepend the data of the new packet in the queue with the packet's index,
        | // a.k.a. "tracking number".
        | packet_index++;
        | packet_queue[queue_head][0] = single(packet_index);
        | //identify the packet version
        | packet_queue[queue_head][1] = -10;
        |
        | // Copy the new packet into the packet_queue.
        | CopyInput();
        |
        | // Increment the head pointer of the packet_queue for the next packet.
        | queue_head = fmod(queue_head + 1, packet_queue_sz);
        | }
    (junction 105) -> AddPacketToQueue : {TrackQueueSize();}
    (junction 104) -> (junction 106) [order 2]
    (junction 104) -> (junction 106) [order 1] : [packet_index == max_packet_id]
        | {packet_index = 0;}
    (junction 106) -> (junction 105) [order 2]
    (junction 106) -> (junction 105) [order 1] : [ queue_head == queue_tail]
        | {queue_tail = fmod(queue_tail + 1, packet_queue_sz);}
  state TrackQueueSize [function]
    (default) -> (junction 114)
    (junction 114) -> (junction 115) [order 1] : [queue_head < queue_tail]
        | { queue_size = queue_head + packet_queue_sz - queue_tail; }
    (junction 114) -> (junction 115) [order 2] : [queue_head >= queue_tail]
        | { queue_size = queue_head - queue_tail; }
  state CopyInput [function]
    (default) -> (junction 119) : { i = 0; }
    (junction 119) -> (junction 119) [order 1] : [i < 300]
        | {
        | packet_queue[queue_head][i + 4] = data_in[i];
        | i++;
        | }
    (junction 119) -> (junction 120) [order 2] : { packet_queue[queue_head][i + 4] = 0.0; }
  state CopyOutput(src_index) [function]
    (default) -> (junction 125) : { i = 0; }
    (junction 125) -> (junction 125) [order 1] : [i < 305]
        | {
        | data_out[i] = packet_queue[src_index][i];
        | i++;
        | }
    (junction 125) -> (junction 126) [order 2]
  data: src_index function_input double; data_out output single size=306; data_in input single size=300; packet_queue local single size=[50000 305]; queue_tail local uint32 =0; queue_head local uint32 =0; queue_size output double =0; total_timeouts output double =0; packet_index local uint32 =0; outstanding_packet_index local uint32; ack_packet_index input uint32; ack_received_flag input double; packet_queue_sz local uint32 =50000; i local uint32; is_task_running input uint8; max_packet_id input uint32
  events: e_send output FUNCTION_CALL_EVENT; e_data_ready_strobe input RISING_EDGE_EVENT; e_clock input EITHER_EDGE_EVENT

== matlab function DataLogging/Poll KINARM/DPRAM Access Subsystem/TypeCast ==
  data: u input double; y output double
function y = fcn(u)

% EML determines output class and size based on first usage
% for some reason the typecast is not setting it correctly, so we 
% explicitly define it first.
y = single(0);

% in order for the typecast to work, both temp and y must be 32 bit
temp = cast(u, 'uint32');
y = typecast(temp, 'single');

== matlab function DataLogging/Poll Force Plates/plate1/parse packet 1 ==
  data: packet input double; forces output double; moments output double; timer output double; calibration input double; gain input double; ain_slope input double; ain_offset input double; orientation input double; zero_voltage input double
function [forces, moments, timer] = fcn(packet, calibration, gain, ain_slope, ain_offset, orientation, zero_voltage)
    %This pulls voltages and timer infomation from the packet we got back from
    %the lab jack.
    
    voltages = zeros(1, 8);
    timers = zeros(1, 3);
    
    for n = 1:8
        bits = readUShort(packet, 13 + ((n - 1)*2));
        voltages(n) = binaryToCalibratedAnalogVoltage(bits, ain_slope, ain_offset);
    end
    
    for n = 1:3
        timers(n) = readUInt(packet, 53 + ((n - 1)*4));
    end
    
    %convert the time stamp to a time in seconds.
    timer = timers(1) / 750000.0; 
    
    %all voltages are between -2.5 to 2.5, here we are normalizeing what we read to zero.
    voltages = voltages - zero_voltage;
    voltages = voltages(1:8); % only the first 8 channels matter.
    
    %using the calibration matrix we convert the to the forces and moments
    values = calibration * (voltages / gain)';
    forces = values(1:3);
    moments = values(4:6);
    
	%reverse the Z force to get it into global coordinates.
	forces(3) = -forces(3);
	
	%considering the positions of the cables push all measures into global coordinates
    if orientation == 0
        forces(2) = -forces(2);
        moments(2) = -moments(2);
    elseif orientation == 90
        y = forces(2);
        forces(2) = -forces(1);
        forces(1) = -y;

        y = moments(2);
        moments(2) = -moments(1);
        moments(1) = -y;
	elseif orientation == 180
        forces(1) = -forces(1);        
        moments(1) = -moments(1);        
    elseif orientation == 270
        y = forces(2);
        forces(2) = forces(1);
        forces(1) = y;

		y = moments(2);
        moments(2) = moments(1);
        moments(1) = y;
    end
end

function val = readUShort(data, offset)
    p1 = uint32(data(offset));
    p2 = uint32(data(offset + 1));
    val = double(p1 + (p2 * 256));
end

function val = readUInt(data, offset)
    p1 = uint32(data(offset));
    p2 = uint32(data(offset + 1));
    p3 = uint32(data(offset + 2));
    p4 = uint32(data(offset + 3));
    val = double(p1 + (p2 * 256) + (p3 * 2^16) + (p4 * 2^24));
end

function voltage = binaryToCalibratedAnalogVoltage(bits, ain_slope, ain_offset)
    voltage = (bits * ain_slope) + ain_offset;
end
